simulink model "e11_pmsm_nonlin_fwc"  (R2024b)
settings: Solver=ode23tb  StartTime=0.0  StopTime=2  MaxStep=0.0001  RelTol=1e-3  EnableMultiTasking=on
InitFcn:
  | d = fileparts(mfilename('fullpath')); while ~exist(fullfile(d, 'models', 'matlab', 'mcb_e11_nonlin_setup.m'), 'file') up = fileparts(d); if strcmp(up, d), break; end, d = up; end, run(fullfile(d, 'models', 'matlab', 'mcb_e11_nonlin_setup.m'));
model workspace (MAT data in the model file):
  encoderResolution = 2000
  hallOffset = '0.5'
  indexOffset = 850
  polePairs = '4'
undefined symbols (not defined in the file): PI_params, pmsm, PU_System, PWM_frequency, Ts, Ts_motor, Ts_speed
libraries: nesl_utility x11, mcbcontrolslib x9, fl_lib x8, ee_lib x7, slpidlib x3, mcbpmsmnonlinearlib x3, mcbpositiondecoderlib x2, nesl_utility_internal x2, simulink x1, eeGeneralControl x1, mcbutilslib x1
(part 1 of 2)
settings Model: Creator=The MathWorks, Inc.  LastModifiedBy=xlin
settings SolverCC: AlgebraicLoopSolver=TrustRegion  MaxZcPerStep=1
settings DataIOCC: LimitDataPoints=on  SaveFormat=Array  SaveOutput=off  SaveTime=off  ReturnWorkspaceOutputs=off
settings OptimizationCC: DefaultParameterBehavior=Inlined  DefaultUnderspecifiedDataType=single  OptimizeBlockIOStorage=off  ReuseModelBlockBuffer=off  EnhancedBackFolding=on  ExpressionDepthLimit=2147483647  ZeroExternalMemoryAtStartup=off  InitFltsAndDblsToZero=on  NoFixptDivByZeroProtection=on  EfficientFloat2IntCast=on  EfficientMapNaN2IntZero=off  LifeSpan=Inf  MaxStackSize=64  DifferentSizesBufferReuse=on  EfficientTunableParamExpr=on
settings DebuggingCC: ReadBeforeWriteMsg=DisableAll  WriteAfterWriteMsg=DisableAll  WriteAfterReadMsg=DisableAll  CheckSSInitialOutputMsg=off  SignalResolutionControl=TryResolveAllWithWarning  SolverPrmCheckMsg=warning  InheritedTsInSrcMsg=none  MultiTaskDSMMsg=none  MultiTaskCondExecSysMsg=none  TasksWithSamePriorityMsg=none  SigSpecEnsureSampleTimeMsg=none  IntegerOverflowMsg=none  ParameterPrecisionLossMsg=none  FcnCallInpInsideContextMsg=warning  UnconnectedInputMsg=warning  UnconnectedOutputMsg=warning  UnconnectedLineMsg=warning  AllowSymbolicDim=off  StateNameClashWarn=warning  SFUnexpectedBacktrackingDiag=warning  SFNoUnconditionalDefaultTransitionDiag=warning  SFExecutionAtInitializationDiag=none  IntegerSaturationMsg=none  ArithmeticOperatorsInVariantConditions=warning
settings HardwareCC: TargetBitPerChar=16  TargetBitPerInt=16  TargetBitPerPointer=16  TargetLargestAtomicInteger=Integer  TargetIntDivRoundTo=Zero  TargetEndianess=LittleEndian  TargetWordSize=16  TargetHWDeviceType=TI C2000
settings ModelReferenceCC: EnableRefExpFcnMdlSchedulingChecks=on  ModelReferenceNumInstancesAllowed=Single  PropagateSignalLabelsOutOfModel=off
settings SFSimCC: SimUseLocalCustomCode=off  MATLABDynamicMemAlloc=off  CustomCodeUndefinedFunction=UseInterfaceOnly
settings RTWCC: Description=Embedded Coder  SystemTargetFile=ert.tlc  TemplateMakefile=ert_default_tmf  GenerateReport=on  RTWUseLocalCustomCode=off  CustomHeaderCode="#include \"F2837xD_Ipc_drivers.h\""  Toolchain=Texas Instruments Code Composer Studio (C2000)  LaunchReport=on  GPUComputeCapability=3.5  DLArmComputeVersion=19.05
settings CodeAppCC: ForceParamTrailComments=on  IgnoreCustomStorageClasses=off  OperatorAnnotations=on  SimulinkDataObjDesc=on  SFDataObjDesc=on  InsertBlockDesc=on  InternalIdentifier=Classic
settings ERTTargetCC: ExtModeStaticAlloc=on  ExtModeStaticAllocSize=10000  ERTCustomFileTemplate=example_file_process.tlc  SuppressUnreachableDefaultCases=off  DynamicArrayContainerType=coder::array
settings ConfigComp: CovMetricSettings=dw  CovSaveCumulativeToWorkspaceVar=on  CovSaveSingleToWorkspaceVar=on  CovExternalEMLEnable=off  CovSFcnEnable=off

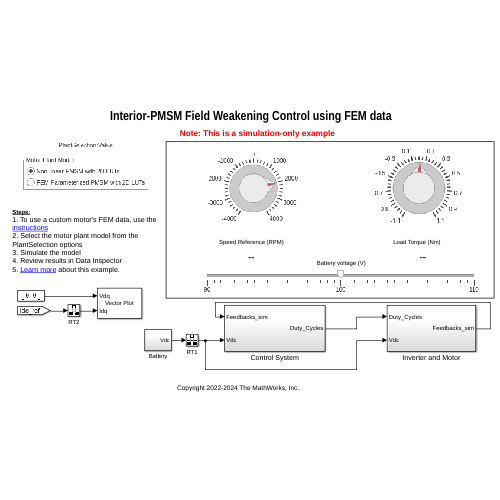
[thumbnail: Simulink's stored preview of the top-level diagram]
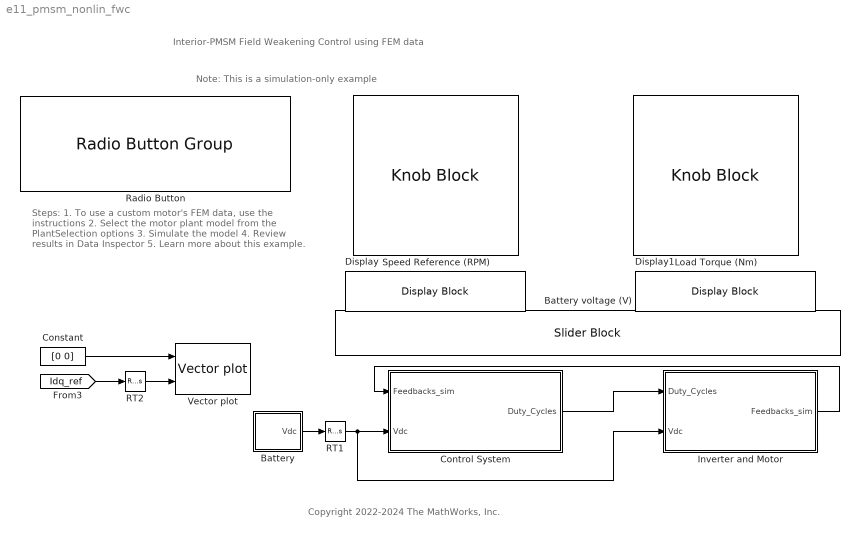
== system e11_pmsm_nonlin_fwc ==
  note: Steps:
      | 1. To use a custom motor's FEM data, use the instructions
      | 2. Select the motor plant model from the PlantSelection options
      | 3. Simulate the model
      | 4. Review results in Data Inspector
      | 5. Learn more about this example.
  note: Copyright 2022-2024 The MathWorks, Inc.
  note: Note: This is a simulation-only example
  note: Interior-PMSM Field Weakening Control using FEM data
  Battery : Subsystem
  Battery voltage (V) : SliderBlock  LabelPosition=Hide  ScaleMin=90  ScaleMax=110  TickInterval=10
  Constant : Constant  Value=[0 0]
  Control System : Subsystem
  Display : DisplayBlock  LabelPosition=Hide  Format=Integer  Transparency=1
  Display1 : DisplayBlock  LabelPosition=Hide  Transparency=1
  Inverter and Motor : Subsystem
  Load Torque (Nm) : KnobBlock  LabelPosition=Hide  ScaleMin=-1.1  ScaleMax=1.1
  RT1 : RateTransition  Deterministic=off  OutPortSampleTime=Ts
  RT2 : RateTransition  Deterministic=off  OutPortSampleTime=0.01
  Radio Button : RadioButtonGroup  SelectedLabel=Non-linear PMSM with 2D LUTs  ButtonGroupName=Motor Plant Model
      settings: Values={{'Non-linear PMSM with 2D LUTs', 'FEM Parameterized PMSM with 2D LUTs'}, [0 1]}
  Speed Reference (RPM) : KnobBlock  LabelPosition=Hide  ScaleMin=-4000  ScaleMax=4000
  Vector plot : mcbutilslib/Vector plot  InputSignals=Vdq Idq  ReferenceFrame=Rotating Reference Frame  axisAlign=D-axis  thetaUnits=Radians  angleUnits=Radians  OpenFigAtSimStart=off  debugEnable=0
      settings: LibrarySourceBlock=mcblib/Signal Management/Vector plot
  wires:
  Control System/1(Duty_Cycles) -> Inverter and Motor/1(Duty_Cycles)
  Constant/1 -> Vector plot/1
  [Idq_ref] -> RT2/1
  RT2/1 -> Vector plot/2
  Inverter and Motor/1(Feedbacks_sim) -> Control System/1(Feedbacks_sim)
  RT1/1 -> Inverter and Motor/2(Vdc), Control System/2(Vdc)
  Battery/1(Vdc) -> RT1/1

== system e11_pmsm_nonlin_fwc/Battery ==
  Battery Voltage : Constant  Value=100
  Vdc : Outport
  wires:
  Battery Voltage/1 -> Vdc/1

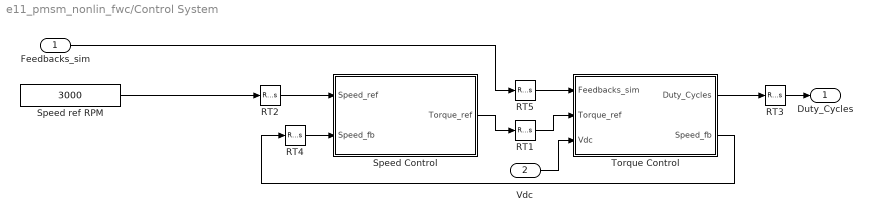
== system e11_pmsm_nonlin_fwc/Control System ==
  Feedbacks_sim : Inport
  Vdc : Inport  Port=2
  RT1 : RateTransition  Deterministic=off  OutPortSampleTime=Ts
  RT2 : RateTransition  Deterministic=off  OutPortSampleTime=Ts_speed
  RT3 : RateTransition  Deterministic=off
  RT4 : RateTransition  Deterministic=off  OutPortSampleTime=Ts_speed
  RT5 : RateTransition  Deterministic=off  OutPortSampleTime=Ts
  Speed Control : Subsystem  TreatAsAtomicUnit=on  SystemSampleTime=Ts_speed
      settings: RTWSystemCode=Nonreusable function
  Speed ref RPM : Constant  Value=3000  OutDataTypeStr=Inherit: Inherit via back propagation  SampleTime=-1
  Torque Control : Subsystem
      settings: RTWSystemCode=Nonreusable function
  Duty_Cycles : Outport
  wires:
  Feedbacks_sim/1 -> RT5/1
  Torque Control/2(Speed_fb) -> RT4/1
  RT1/1 -> Torque Control/2(Torque_ref)
  Speed Control/1(Torque_ref) -> RT1/1
  RT5/1 -> Torque Control/1(Feedbacks_sim)
  RT4/1 -> Speed Control/2(Speed_fb)
  Torque Control/1(Duty_Cycles) -> RT3/1
  RT2/1 -> Speed Control/1(Speed_ref)
  RT3/1 -> Duty_Cycles/1
  Vdc/1 -> Torque Control/3(Vdc)
  Speed ref RPM/1 -> RT2/1

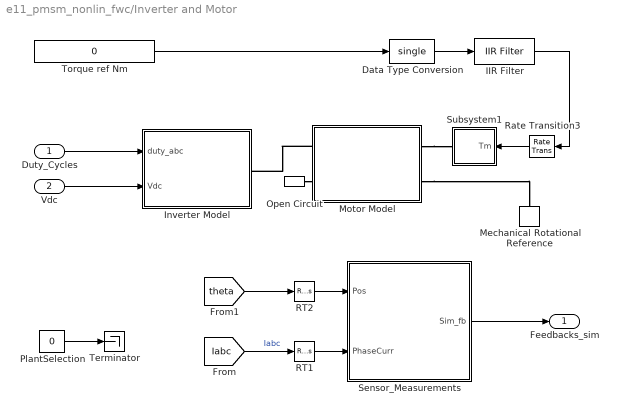
== system e11_pmsm_nonlin_fwc/Inverter and Motor ==
  Duty_Cycles : Inport
  Vdc : Inport  Port=2
  Data Type Conversion : DataTypeConversion  OutDataTypeStr=single  SaturateOnIntegerOverflow=off  RndMeth=Floor
  IIR Filter : mcbcontrolslib/IIR Filter  VariantControl=Low Pass Filter  VariantSelect=Low-pass  FilterConstantInputType=Specify via dialog  Filter_constant=0.01  advancedSettings=off  Ts=50e-6  cutOff_freq=32.1525
  Inverter Model : Subsystem
  Mechanical Rotational Reference : fl_lib/Mechanical/Rotational Elements/Mechanical Rotational Reference
  Motor Model : Subsystem  Variant=on
  Open Circuit : fl_lib/Electrical/Electrical Elements/Open Circuit  v_specify=off  v_priority=None  v=0 V  v_nominal_specify=off  v_nominal_value=1  v_nominal_unit=V
  PlantSelection : Constant  Value=0
  RT1 : RateTransition  Deterministic=off  OutPortSampleTime=Ts_simulink
  RT2 : RateTransition  Deterministic=off  OutPortSampleTime=Ts_simulink
  Rate Transition3 : RateTransition  Deterministic=off  OutPortSampleTime=Ts_motor
  Sensor_Measurements : Subsystem
  Subsystem1 : Subsystem
  Terminator : Terminator
  Torque ref Nm : Constant  Value=0  OutDataTypeStr=dataType  SampleTime=-1
  Feedbacks_sim : Outport  VectorParamsAs1DForOutWhenUnconnected=off
  wires:
  Sensor_Measurements/1(Sim_fb) -> Feedbacks_sim/1
  Torque ref Nm/1 -> Data Type Conversion/1
  Data Type Conversion/1 -> IIR Filter/1
  IIR Filter/1 -> Rate Transition3/1
  RT2/1 -> Sensor_Measurements/1(Pos)
  Rate Transition3/1 -> Subsystem1/1(Tm)
  [theta] -> RT2/1
  RT1/1 -> Sensor_Measurements/2(PhaseCurr)
  [Iabc] -> RT1/1  "Iabc"
  Duty_Cycles/1 -> Inverter Model/1(duty_abc)
  PlantSelection/1 -> Terminator/1
  Vdc/1 -> Inverter Model/2(Vdc)
  connections:
  Open Circuit/LConn1 -- Motor Model/LConn2
  Motor Model/RConn2 -- Mechanical Rotational Reference/LConn1
  Motor Model/RConn1 -- Subsystem1/RConn1
  Motor Model/LConn1 -- Inverter Model/RConn1

== system e11_pmsm_nonlin_fwc/Control System/Speed Control ==
  Speed_ref : Inport
  Speed_fb : Inport  Port=2
  PI_Controller_Speed : Subsystem
  rpm2pu : Subsystem
  Torque_ref : Outport  VectorParamsAs1DForOutWhenUnconnected=off
  wires:
  Speed_ref/1 -> rpm2pu/1(In1)  "speed_ref_rpm"
  Speed_fb/1 -> PI_Controller_Speed/2(Speed_fb)  "speed_fb"
  PI_Controller_Speed/1(T_ref) -> Torque_ref/1
  rpm2pu/1(Speed_ref) -> PI_Controller_Speed/1(Speed_ref)  "speed_ref"

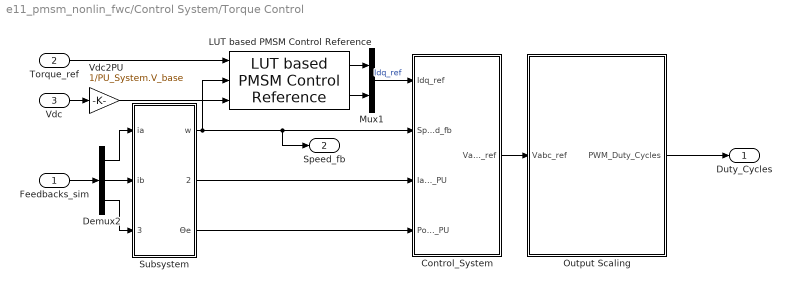
== system e11_pmsm_nonlin_fwc/Control System/Torque Control ==
  Feedbacks_sim : Inport
  Torque_ref : Inport  Port=2
  Vdc : Inport  Port=3
  Control_System : Subsystem
  Demux2 : Demux  Outputs=3
  LUT based PMSM Control Reference : mcbpmsmnonlinearlib/LUT based PMSM Control Reference  motorType=Interior PMSM  FWCMethod=CVCP  polePairs=pmsm.p  Rs=pmsm.Rs  nonLinearityChoice=Non-linear model with id and iq LUTs  Ld=pmsm.Ld  Lq=pmsm.Lq  FluxPM=pmsm.FluxPM  Vdc_input_select=Input port - use 2D LUT (scaled-w based)  vdc=inverter.V_dc  vdcVec=[18 30]  idVec=PMSMLUT.idVec  iqVec=PMSMLUT.iqVec  LdTable=PMSMLUT.LdTable  LqTable=PMSMLUT.LqTable  FluxPMTable=PMSMLUT.FluxPMTable  FluxDTable=[-1.6,-1.6,-1.6,-1.6,-1.6;2.4,2.4,2.4,2.4,2.4;6.4,6.4,6.4,6.4,6.4;10.4,10.4,10.4,10.4,10.4]*1e-3  FluxQTable=[-8,-4,0,4,8;-8,-4,0,4,8;-8,-4,0,4,8;-8,-4,0,4,8]*1e-3  useMeasTorqTable=off  MeasuredTorqTable=[-3.4560,-1.7280,0, 1.7280, 3.4560;-2.4960,-1.2480,0, 1.2480, 2.4960;-1.5360,-0.7680,0, 0.7680, 1.5360;-0.5760,-0.2880,0, 0.2880, 0.5760]  useTorquePct=off  CustomGrid=off  trefVec=PMSMLUT.trefVec  trefPctVec=[0 50 100]  Tenvelope=[0.3 0.3 0.15 0.05]  wrpmVec=PMSMLUT.wrpmVec  idTable=PMSMLUT.idTable  iqTable=PMSMLUT.iqTable  idTable3d=cat(3,[0,0,0,-7.1;-0.4579,-0.4579,-0.4579,-7.1;-1.4457,-1.4457,-1.4457,-7.1],[0,0,0,0;-0.4579,-0.4579,-0.4579,-1.2581;-1.4457,-1.4457,-1.4457,-4.5085])  iqTable3d=cat(3,[0,0,0,0;3.8539,3.8539,3.8539,0;6.9513,6.9513,6.9513,0],[0,0,0,0;3.8539,3.8539,3.8539,3.7611;6.9513,6.9513,6.9513,5.4848])  ilimit=maxMotorCurrent  Bv=pmsm.B  Units=Per-Unit (PU)  V_base=PU_System.V_base  I_base=PU_System.I_base  N_base=pmsm.N_base  T_base=0.74112  scaledTables=on  saveLUTs=off  useDefaultPlotOptions=on  RPM2plot=3000  Torque2plot=0.1  driveChar2plot=off  enableiMax2plot=off  imax2plot=10
      settings: LibrarySourceBlock=mcblib/Controls/Control Reference/LUT based PMSM Control Reference
  Mux1 : Mux  Inputs=2
  Output Scaling : Subsystem
  Subsystem : Subsystem
  Vdc2PU : Gain  Gain=1/PU_System.V_base  RndMeth=Simplest  OutDataTypeStr=Inherit: Same as input
  Duty_Cycles : Outport  InitialOutput=0  VectorParamsAs1DForOutWhenUnconnected=off
  Speed_fb : Outport  Port=2  InitialOutput=0  VectorParamsAs1DForOutWhenUnconnected=off
  wires:
  Control_System/1(Vabc_ref) -> Output Scaling/1(Vabc_ref)
  Output Scaling/1(PWM_Duty_Cycles) -> Duty_Cycles/1
  Feedbacks_sim/1 -> Demux2/1
  Subsystem/1(w) -> Speed_fb/1, Control_System/2(Speed_fb), LUT based PMSM Control Reference/2
  Demux2/1 -> Subsystem/1(ia)
  Demux2/2 -> Subsystem/2(ib)
  Demux2/3 -> Subsystem/3(pos_rad)
  Subsystem/2(iab_pu) -> Control_System/3(Iab_meas_PU)
  Subsystem/3(ϴe) -> Control_System/4(Pos_meas_PU)
  LUT based PMSM Control Reference/1 -> Mux1/1
  LUT based PMSM Control Reference/2 -> Mux1/2
  Mux1/1 -> Control_System/1(Idq_ref)  "Idq_ref"
  Torque_ref/1 -> LUT based PMSM Control Reference/1
  Vdc/1 -> Vdc2PU/1
  Vdc2PU/1 -> LUT based PMSM Control Reference/3

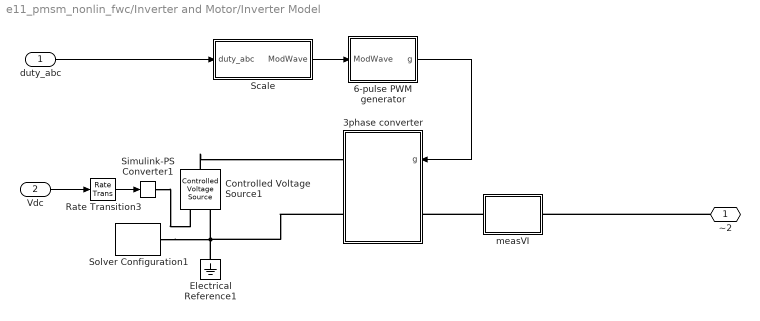
== system e11_pmsm_nonlin_fwc/Inverter and Motor/Inverter Model ==
  duty_abc : Inport
  Vdc : Inport  Port=2
  3phase converter : Subsystem
  6-pulse PWM generator : Subsystem  mask{fs=PWM_frequency}
      mask prompts: fs "Carrier Frequency (Hz)"
  Controlled Voltage Source1 : fl_lib/Electrical/Electrical Sources/Controlled Voltage Source
  Electrical Reference1 : fl_lib/Electrical/Electrical Elements/Electrical Reference
  Rate Transition3 : RateTransition  Deterministic=off  OutPortSampleTime=Ts_motor
  Scale : Subsystem
  Simulink-PS Converter1 : nesl_utility/Simulink-PS Converter  PhysicalDomain=network_engine_domain  SubClassName=ps_input  LeftPortType=input  RightPortType=output  PseudoPeriodic=off  Frequencies=[]  NoiseDistribution=none  NoiseParameters=[]  Unit=1  AffineConversion=off  FilteringAndDerivatives=provide  SimscapeFilterOrder=1  InputFilterTimeConstant=0.001  UdotUserProvided=0
  Solver Configuration1 : nesl_utility/Solver Configuration  PhysicalDomain=network_engine_domain  SubClassName=solver  LeftPortType=input  RightPortType=generic  Tones=[]  Harmonics=[]  SimulateNoise=off  Profile=off  UseLocalSampling=off  EnableSwitchedLinearOptims=on  FrequencyDomain=off  UseCCode=off  RelTol=0.001  AbsTol=0.001  MinStep=1e-09  ToWorkspace=off  RevertToSquareIcSolve=off  NumHomotopyIterations=100  PhasorMode=off  PhasorModeNumHarmonics=1  ConsistencySolver=NEWTON_XTOL_AFTER_FTOL  IndexReductionMethod=DerivativeReplacement  DoDC=off  ResidualTolerance=1e-09  ConsistencyTolSource=GLOBAL  ConsistencyAbsTol=0.001  ConsistencyRelTol=0.001  ConsistencyTolFactor=1e-09  UseLocalSolver=on  LocalSolverChoice=NE_BACKWARD_EULER_ADVANCER  ResolveIndetEquations=on  FunctionEvalNumThread=1  LocalSolverSampleTime=Ts_motor  DoFixedCost=on  MaxNonlinIter=1  MaxModeIter=2  ComputeImpulses=off  ImpulseIterations=2  LinearAlgebra=Sparse  LinearAlgebraNumThread=0  EquationFormulation=NE_TIME_EF  DelaysMemoryBudget=1024  AutomaticFiltering=off  FilteringTimeConstant=0.001  PartitionStorageMethod=AS_NEEDED  PartitionMemoryBudget=1024  PartitionMethod=ROBUST  MultibodyUseLocalSolver=off  MultibodyLocalSolverChoice=ODE1  MultibodyLocalSolverSampleTime=0.001
  measVI : Subsystem
  ~2 : PMIOPort  Side=Right
  wires:
  6-pulse PWM generator/1(g) -> 3phase converter/1(g)
  duty_abc/1 -> Scale/1(duty_abc)
  Scale/1(ModWave) -> 6-pulse PWM generator/1(ModWave)
  Rate Transition3/1 -> Simulink-PS Converter1/1
  Vdc/1 -> Rate Transition3/1
  connections:
  measVI/LConn1 -- 3phase converter/LConn1
  Electrical Reference1/LConn1 -- Solver Configuration1/RConn1 -- 3phase converter/RConn2 -- Controlled Voltage Source1/RConn2
  Controlled Voltage Source1/LConn1 -- 3phase converter/RConn1
  ~2/RConn1 -- measVI/RConn1
  Simulink-PS Converter1/RConn1 -- Controlled Voltage Source1/RConn1

== system e11_pmsm_nonlin_fwc/Inverter and Motor/Motor Model ==
  FEM Parameterized PMSM 2D LUTs : Subsystem  VariantControl=(get_param([bdroot '/Inverter and Motor/PlantSelection'], 'Value') == '1')
  Non-linear PMSM with 2D LUTs : Subsystem  VariantControl=(get_param([bdroot '/Inverter and Motor/PlantSelection'], 'Value') == '0')
  ~ : PMIOPort  Side=Left
  neutral : PMIOPort  Port=2  Side=Left
  R : PMIOPort  Port=3  Side=Right
  C : PMIOPort  Port=4  Side=Right

== system e11_pmsm_nonlin_fwc/Inverter and Motor/Sensor_Measurements ==
  Pos : Inport
  PhaseCurr : Inport  Port=2
  Data Type Conversion2 : DataTypeConversion  OutDataTypeStr=single  RndMeth=Simplest  SaturateOnIntegerOverflow=off
  Data Type Conversion4 : DataTypeConversion  OutDataTypeStr=single  RndMeth=Simplest  SaturateOnIntegerOverflow=off
  Delay1 : Delay  DelayLength=PI_params.delay_Currents
  Delay2 : Delay  DelayLength=PI_params.delay_Position
  Mux2 : Mux  Inputs=2
  Selector : Selector  InputPortWidth=3  IndexOptions=Index vector (dialog)  Indices=[1 2]  OutputSizes=1
  Sim_fb : Outport  VectorParamsAs1DForOutWhenUnconnected=off
  wires:
  Delay1/1 -> Selector/1  "Iab_fb"
  Data Type Conversion4/1 -> Delay1/1
  PhaseCurr/1 -> Data Type Conversion4/1
  Pos/1 -> Data Type Conversion2/1
  Data Type Conversion2/1 -> Delay2/1  "Theta_m"
  Selector/1 -> Mux2/1
  Delay2/1 -> Mux2/2  "Theta_m"
  Mux2/1 -> Sim_fb/1

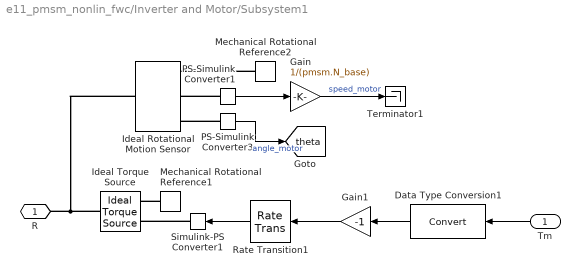
== system e11_pmsm_nonlin_fwc/Inverter and Motor/Subsystem1 ==
  Tm : Inport
  Data Type Conversion1 : DataTypeConversion  SaturateOnIntegerOverflow=off  RndMeth=Floor
  Gain : Gain  Gain=1/(pmsm.N_base)
  Gain1 : Gain  Gain=-1
  Ideal Rotational Motion Sensor : fl_lib/Mechanical/Mechanical Sensors/Ideal Rotational Motion Sensor  reference=foundation.enum.MeasurementReference.difference  acceleration_port=false  velocity_port=true  position_port=true  wrap_angle=simscape.enum.onoff.off  offset=0 rad
  Ideal Torque Source : fl_lib/Mechanical/Mechanical Sources/Ideal Torque Source
  Mechanical Rotational Reference1 : fl_lib/Mechanical/Rotational Elements/Mechanical Rotational Reference
  Mechanical Rotational Reference2 : fl_lib/Mechanical/Rotational Elements/Mechanical Rotational Reference
  PS-Simulink Converter1 : nesl_utility/PS-Simulink Converter  PhysicalDomain=network_engine_domain  SubClassName=ps_output  LeftPortType=input  RightPortType=output  PseudoPeriodic=off  Frequencies=[]  VectorFormat=inherit  Unit=inherit  AffineConversion=off
  PS-Simulink Converter3 : nesl_utility/PS-Simulink Converter  PhysicalDomain=network_engine_domain  SubClassName=ps_output  LeftPortType=input  RightPortType=output  PseudoPeriodic=off  Frequencies=[]  VectorFormat=inherit  Unit=inherit  AffineConversion=off
  Rate Transition1 : RateTransition
  Simulink-PS Converter1 : nesl_utility/Simulink-PS Converter  PhysicalDomain=network_engine_domain  SubClassName=ps_input  LeftPortType=input  RightPortType=output  PseudoPeriodic=off  Frequencies=[]  NoiseDistribution=none  NoiseParameters=[]  Unit=1  AffineConversion=off  FilteringAndDerivatives=provide  SimscapeFilterOrder=1  InputFilterTimeConstant=0.001  UdotUserProvided=0
  Terminator1 : Terminator
  "R " : PMIOPort  Side=Right
  tag scope: theta=global
  wires:
  Gain1/1 -> Rate Transition1/1
  Rate Transition1/1 -> Simulink-PS Converter1/1
  Data Type Conversion1/1 -> Gain1/1
  Tm/1 -> Data Type Conversion1/1
  PS-Simulink Converter1/1 -> Gain/1
  Gain/1 -> Terminator1/1  "speed_motor"
  PS-Simulink Converter3/1 -> [theta]  "angle_motor"
  connections:
  Mechanical Rotational Reference1/LConn1 -- Ideal Torque Source/RConn2
  Simulink-PS Converter1/RConn1 -- Ideal Torque Source/RConn1
  Ideal Torque Source/LConn1 -- Ideal Rotational Motion Sensor/LConn1 -- "R "/RConn1
  PS-Simulink Converter1/LConn1 -- Ideal Rotational Motion Sensor/RConn2
  PS-Simulink Converter3/LConn1 -- Ideal Rotational Motion Sensor/RConn3
  Mechanical Rotational Reference2/LConn1 -- Ideal Rotational Motion Sensor/RConn1

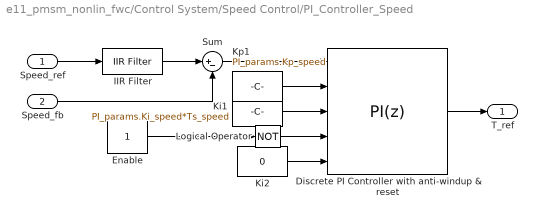
== system e11_pmsm_nonlin_fwc/Control System/Speed Control/PI_Controller_Speed ==
  Speed_ref : Inport
  Speed_fb : Inport  Port=2
  Discrete PI Controller with anti-windup & reset : slpidlib/PID Controller  Controller=PI  Form=Parallel  TimeDomain=Discrete-time  UseExternalTs=off  SampleTime=-1  IntegratorMethod=Forward Euler  FilterMethod=Forward Euler  ControllerParametersSource=external  P=1  I=1  UseKiTs=on  D=0  UseExternalDerivativeSource=off  N=100  UseFilter=on  TunerSelectOption=Transfer Function Based (PID Tuner App)  InitialConditionSource=external  InitialConditionForIntegrator=0  InitialConditionForFilter=0  DifferentiatorICPrevScaledInput=0  ExternalReset=level  TrackingMode=off  Kt=1  LimitOutput=on  SatLimitsSource=internal  UpperSaturationLimit=1  LowerSaturationLimit=-1  LinearizeAsGain=on  AntiWindupMode=clamping  Kb=1  LimitIntegrator=off  UpperIntegratorSaturationLimit=inf  LowerIntegratorSaturationLimit=-inf  RndMeth=Simplest  POutMin=[]  POutMax=[]  IOutMin=[]  IOutMax=[]  DOutMin=[]  DOutMax=[]  NOutMin=[]  NOutMax=[]  SumOutMin=[]  SumOutMax=[]  SaturationOutDataTypeStr=Inherit: Inherit via back propagation  SaturationOutMin=[]  SaturationOutMax=[]  PParamMin=[]  PParamMax=[]  IParamMin=[]  IParamMax=[]  DParamMin=[]  DParamMax=[]  NParamMin=[]  NParamMax=[]  KbParamMin=[]  KbParamMax=[]  KtParamMin=[]  KtParamMax=[]  KbOutMin=[]  KbOutMax=[]  KtOutMin=[]  KtOutMax=[]  IntegratorOutMin=[]  IntegratorOutMax=[]  FilterOutMin=[]  FilterOutMax=[]  SumI1OutMin=[]  SumI1OutMax=[]  SumI2OutMin=[]  SumI2OutMax=[]  SumI3OutMin=[]  SumI3OutMax=[]  SumI4OutMin=[]  SumI4OutMax=[]  SumDOutMin=[]  SumDOutMax=[]  DifferentiatorOutMin=[]  DifferentiatorOutMax=[]  FilterDiffOutCoefMin=[]  FilterDiffOutCoefMax=[]  ReciprocalOutMin=[]  ReciprocalOutMax=[]  SumDenOutMin=[]  SumDenOutMax=[]  SumNumOutMin=[]  SumNumOutMax=[]  DivideOutMin=[]  DivideOutMax=[]  UdiffTsProdOutMin=[]  UdiffTsProdOutMax=[]  NTsProdOutMin=[]  NTsProdOutMax=[]  UintegralTsProdOutMin=[]  UintegralTsProdOutMax=[]  UngainTsProdOutMin=[]  UngainTsProdOutMax=[]  ClampingZeroOutDataTypeStr=Inherit: Inherit via back propagation  ClampingZeroOutMin=[]  ClampingZeroOutMax=[]  FilterDenConstantOutDataTypeStr=Inherit: Inherit via back propagation  FilterDenConstantOutMin=[]  FilterDenConstantOutMax=[]  PCopyOutDataTypeStr=Inherit: Inherit via back propagation  PCopyOutMin=[]  PCopyOutMax=[]  NCopyOutDataTypeStr=Inherit: Inherit via back propagation  NCopyOutMin=[]  NCopyOutMax=[]  IntegratorContinuousStateAttributes=''  IntegratorStateMustResolveToSignalObject=off  IntegratorRTWStateStorageClass=Auto  FilterContinuousStateAttributes=''  FilterStateMustResolveToSignalObject=off  FilterRTWStateStorageClass=Auto  ParallelPVariant=ExternalParameters  IdealPVariant=Disabled  IVariant=ExternalParameters  DVariant=Disabled  IntegratorVariant=Discrete  SatVariant=Enabled  AWVariant=DiscClampingParallel  PCopyVariant=Disabled  TRVariant=Disabled  FdbkBlocksVariant=Forward  IdealPFdbkVariant=Disabled  SatFdbkVariant=Disabled  DerivativeFilterVariant=Disabled  NVariant=Disabled  NCopyVariant=Disabled_SignalSpec  FilterICVariant=Disabled  IntegratorICVariant=ExternalICs  ExternalResetVariant=ExternalReset  TRSumVariant=Passthrough  SumFdbkVariant=Disabled  SumVariant=Sum_PI  TsampFilterVariant=InternalTs  TsampNgainVariant=Passthrough  TsampIntegralVariant=Disabled_SignalSpec  ExternalSaturationOutDataTypeStr=Inherit: Same as second input  DerivativeSourceVariant=Disabled  PreIntVariant=InternalPreInt
  Enable : Constant  OutDataTypeStr=boolean  SampleTime=-1
  IIR Filter : mcbcontrolslib/IIR Filter  VariantControl=Low Pass Filter  VariantSelect=Low-pass  FilterConstantInputType=Specify via dialog  Filter_constant=0.1  advancedSettings=off  Ts=50e-6  cutOff_freq=353.6777
  Ki1 : Constant  Value=PI_params.Ki_speed*Ts_speed  OutDataTypeStr=dataType  SampleTime=-1
  Ki2 : Constant  Value=0  OutDataTypeStr=dataType  SampleTime=-1
  Kp1 : Constant  Value=PI_params.Kp_speed  OutDataTypeStr=dataType  SampleTime=-1
  Logical Operator : Logic  Operator=NOT  IconShape=distinctive  AllPortsSameDT=off  OutDataTypeStr=boolean
  Sum : Sum  Inputs=|+-
  T_ref : Outport  VectorParamsAs1DForOutWhenUnconnected=off
  wires:
  Discrete PI Controller with anti-windup & reset/1 -> T_ref/1
  Ki1/1 -> Discrete PI Controller with anti-windup & reset/3
  Kp1/1 -> Discrete PI Controller with anti-windup & reset/2
  Speed_fb/1 -> Sum/2
  Sum/1 -> Discrete PI Controller with anti-windup & reset/1
  Logical Operator/1 -> Discrete PI Controller with anti-windup & reset/4
  Enable/1 -> Logical Operator/1
  Ki2/1 -> Discrete PI Controller with anti-windup & reset/5
  Speed_ref/1 -> IIR Filter/1
  IIR Filter/1 -> Sum/1

== system e11_pmsm_nonlin_fwc/Control System/Speed Control/rpm2pu ==
  In1 : Inport
  Data Type Conversion2 : DataTypeConversion  OutDataTypeStr=dataType  RndMeth=Simplest  SaturateOnIntegerOverflow=off
  rpm2PU : Gain  Gain=1/pmsm.N_base  RndMeth=Simplest  OutDataTypeStr=Inherit: Same as input
  Speed_ref : Outport
  wires:
  Data Type Conversion2/1 -> Speed_ref/1
  rpm2PU/1 -> Data Type Conversion2/1
  In1/1 -> rpm2PU/1

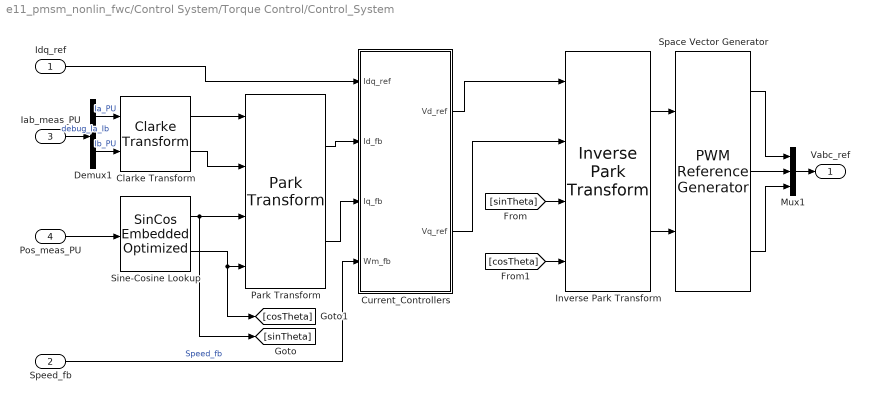
== system e11_pmsm_nonlin_fwc/Control System/Torque Control/Control_System ==
  Idq_ref : Inport
  Speed_fb : Inport  Port=2
  Iab_meas_PU : Inport  Port=3
  Pos_meas_PU : Inport  Port=4
  Clarke Transform : mcbcontrolslib/Clarke Transform  VariantControl=Variant2  PhaseInput=Two inputs  EnPowerInv=off
  Current_Controllers : Subsystem
  Demux1 : Demux  Outputs=2
  Inverse Park Transform : mcbcontrolslib/Inverse Park Transform  PhaseInput=Two inputs  AxisAlignment=D-axis  ThetaInput=Sine and Cosine electrical position  AngleInput=Per-unit  N_points=1024
  Mux1 : Mux  Inputs=3
  Park Transform : mcbcontrolslib/Park Transform  PhaseInput=Two inputs  AxisAlignment=D-axis  ThetaInput=Sine and Cosine electrical position  AngleInput=Per-unit  N_points=1024
  Sine-Cosine Lookup : mcbcontrolslib/SinCos Embedded Optimized  LabelModeActiveChoice=MCB_Sin  OptforProc=off  ApproximationMethod=None  UserApproxMethod=Lookup  ApproxStatus=None  InterpMethod=Linear point-slope  NumberOfDataPoints=16  NumberOfIterations=11  RemoveProtectionAgainstOutOfRangeInput=off  TableDataTypeStr=Inherit: Inherit via input  AngleInput=Per-unit  ThetaDataType=single  N_points=1024  DatatypeInput=Inherit from input  Datatype=single
  Space Vector Generator : mcbcontrolslib/PWM Reference Generator  inSignal=Valphabeta  modType=SVM: space vector modulation
  Vabc_ref : Outport  VectorParamsAs1DForOutWhenUnconnected=off
  wires:
  Park Transform/1 -> Current_Controllers/2(Id_fb)
  Park Transform/2 -> Current_Controllers/3(Iq_fb)
  Inverse Park Transform/1 -> Space Vector Generator/1
  Inverse Park Transform/2 -> Space Vector Generator/2
  Sine-Cosine Lookup/1 -> [sinTheta], Park Transform/3
  Sine-Cosine Lookup/2 -> [cosTheta], Park Transform/4
  [cosTheta] -> Inverse Park Transform/4
  [sinTheta] -> Inverse Park Transform/3
  Clarke Transform/2 -> Park Transform/2
  Clarke Transform/1 -> Park Transform/1
  Idq_ref/1 -> Current_Controllers/1(Idq_ref)
  Space Vector Generator/1 -> Mux1/1
  Space Vector Generator/2 -> Mux1/2
  Current_Controllers/1(Vd_ref) -> Inverse Park Transform/1
  Current_Controllers/2(Vq_ref) -> Inverse Park Transform/2
  Space Vector Generator/3 -> Mux1/3
  Mux1/1 -> Vabc_ref/1
  Demux1/1 -> Clarke Transform/1  "Ia_PU"
  Demux1/2 -> Clarke Transform/2  "Ib_PU"
  Iab_meas_PU/1 -> Demux1/1  "debug_Ia_Ib"
  Speed_fb/1 -> Current_Controllers/4(Wm_fb)  "Speed_fb"
  Pos_meas_PU/1 -> Sine-Cosine Lookup/1

== system e11_pmsm_nonlin_fwc/Control System/Torque Control/Output Scaling ==
  Vabc_ref : Inport
  Constant : Constant  Value=0.5  OutDataTypeStr=dataType  SampleTime=-1
  One_by_Two : Gain  Gain=0.5  RndMeth=Simplest  OutDataTypeStr=Inherit: Same as input
  Sum : Sum  Inputs=|++
  PWM_Duty_Cycles : Outport
  wires:
  Constant/1 -> Sum/2
  Vabc_ref/1 -> One_by_Two/1
  Sum/1 -> PWM_Duty_Cycles/1
  One_by_Two/1 -> Sum/1

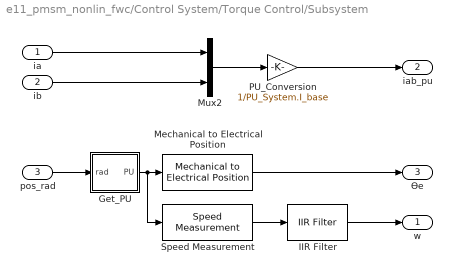
== system e11_pmsm_nonlin_fwc/Control System/Torque Control/Subsystem ==
  ia : Inport
  ib : Inport  Port=2
  pos_rad : Inport  Port=3
  "Get_PU " : Subsystem
  IIR Filter : mcbcontrolslib/IIR Filter  VariantControl=Low Pass Filter  VariantSelect=Low-pass  FilterConstantInputType=Specify via dialog  Filter_constant=IIR_filter_speed.coeff_Ts  advancedSettings=off  Ts=50e-6  cutOff_freq=1
  Mechanical to Electrical Position : mcbpositiondecoderlib/Mechanical to Electrical Position  PolePairsInputType=Specify via dialog  NrPP=pmsm.p  selectedRange=Per unit  MechOfstInputType=Specify via dialog  mechOffsetIn=0  maxAngleIn=1  InputDataType=dataType  VariantSelect=floating-point
  Mux2 : Mux  Inputs=2
  PU_Conversion : Gain  Gain=1/PU_System.I_base  RndMeth=Simplest  OutDataTypeStr=Inherit: Same as input
  Speed Measurement : mcbpositiondecoderlib/Speed Measurement  PositionUnit=Per unit  PositionScalingDatatype=uint32  SpeedCalculationMode=Time interval for speed calculation  SampleTimeAsync=Ts  MaximumApplicationSpeed=6000  SpeedResolution=5e-6  DelayLength=20  MaximumMeasurableSpeed=-0.98352  MeasurableSpeedResolution=7.6757e-12  SpeedUnit=Per unit based on dialog  PerUnitSpeed=PU_System.N_base  SpeedDataType=dataType
  w : Outport
  iab_pu : Outport  Port=2
  ϴe : Outport  Port=3
  wires:
  ib/1 -> Mux2/2
  "Get_PU "/1(PU) -> Speed Measurement/1, Mechanical to Electrical Position/1
  ia/1 -> Mux2/1
  PU_Conversion/1 -> iab_pu/1
  Speed Measurement/1 -> IIR Filter/1
  Mux2/1 -> PU_Conversion/1
  pos_rad/1 -> "Get_PU "/1(rad)
  IIR Filter/1 -> w/1
  Mechanical to Electrical Position/1 -> ϴe/1

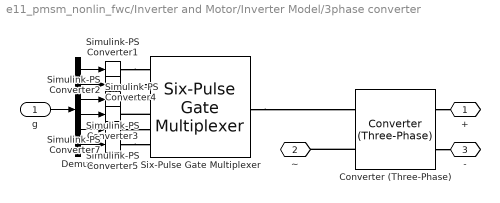
== system e11_pmsm_nonlin_fwc/Inverter and Motor/Inverter Model/3phase converter ==
  g : Inport
  Converter (Three-Phase) : ee_lib/Semiconductors & Converters/Converters/Converter (Three-Phase)  port_option=ee.enum.threePhasePort.composite  fidelity_option=ee.enum.converters.fidelity.detailed  device_type=ee.enum.converters.switchingdevice.ideal  showThermalPort=false  K=0  Vth=0.5 V  Vgt=1 V  Vgt_off=-1 V  Ih=1 A  Vf=0.8 V  Ron=0.001 Ohm  Rds=0.001 Ohm  Goff=1e-6 1/Ohm  Eon_scalar=22.86e-3 J  Eoff_scalar=17.14e-3 J  Eoff_natural_commutation=10e-3 J  Voff=300 V  Iout_scalar=600 A  onCurrentMeasDelay=0 s  useCurrentFromPreviousCycle=false  useVoltageFromPreviousCycle=false  diode_param=ee.enum.converters.protectiondiode.none  diode_Vf=0.8 V  diode_Ron=0.001 Ohm  diode_Goff=1e-5 1/Ohm  diode_C=50 nF  diode_iRM=-235 A  diode_iF=300 A  diode_idot=-50 A/us  diode_trr_param=ee.enum.converters.diodetrr.trr_factor  diode_trr_factor=3  diode_trr=15 us  diode_Qrr=1500 s*uA  diode_rec_loss_model=ee.enum.diode.reverseRecoveryModel.fixed  diode_ErecVal=0 J  diode_scaleWithIandV=false  diode_ErecMat=zeros(2, 3) J  diode_TjrecVec=[298.15, 398.15] K  diode_IfrecVec=[.1, 1, 10] A  diode_IrecVal=10 A  diode_VrecVal=10 V  diode_tFilter=1 / 1000 / 100 s  thermal_network_parameterization=ee.enum.thermalNetworkTopology.external  Rth=[.08, .5] K/W  Rth_Cauer=[.08, .1, .5] K/W  Rth_Foster=[.08, .14, .22, .16] K/W  thermal_mass_parameterization=ee.enum.thermalNetwork.timeconstant  thermal_mass=[.01, .5] J/K  thermal_mass_Cauer=[.01, .1, .5] J/K  thermal_mass_Foster=[.001, .005, .05, .5] J/K  thermal_time_constant=[.001, .2] s  thermal_time_constant_Cauer=[.001, .1, .2] s  thermal_time_constant_Foster=[7e-05, .0007, .01, .08] s  thermal_mass_initial_temperatures=[25, 25] degC  thermal_mass_initial_temperatures_Cauer=[25, 25, 25] degC  junction_thermal_mass=0.01 J/K  Tvec_initial_Foster=[25, 25, 25, 25] degC  snubber_type=ee.enum.converters.snubber.exclude  Cs=1e-7 F  Rs=0.1 Ohm  Vce_loss=[0, 150, 300] V
  Demux : Demux  Outputs=6
  Simulink-PS Converter{1..5,7} (6 alike) : nesl_utility/Simulink-PS Converter  PhysicalDomain=network_engine_domain  SubClassName=ps_input  LeftPortType=input  RightPortType=output  PseudoPeriodic=off  Frequencies=[]  NoiseDistribution=none  NoiseParameters=[]  Unit=1  AffineConversion=off  FilteringAndDerivatives=provide  SimscapeFilterOrder=1  InputFilterTimeConstant=0.001  UdotUserProvided=0
  Six-Pulse Gate Multiplexer : ee_lib/Semiconductors & Converters/Converters/Six-Pulse Gate Multiplexer  port_option=ee.enum.controlport.ps
  + : PMIOPort  Side=Right
  ~ : PMIOPort  Port=2  Side=Left
  - : PMIOPort  Port=3  Side=Right
  wires:
  g/1 -> Demux/1
  Demux/1 -> Simulink-PS Converter1/1
  Demux/2 -> Simulink-PS Converter2/1
  Demux/3 -> Simulink-PS Converter3/1
  Demux/4 -> Simulink-PS Converter4/1
  Demux/6 -> Simulink-PS Converter7/1
  Demux/5 -> Simulink-PS Converter5/1
  connections:
  Simulink-PS Converter1/RConn1 -- Six-Pulse Gate Multiplexer/LConn1
  Converter (Three-Phase)/RConn2 -- -/RConn1
  Converter (Three-Phase)/RConn1 -- +/RConn1
  Converter (Three-Phase)/LConn2 -- ~/RConn1
  Six-Pulse Gate Multiplexer/RConn1 -- Converter (Three-Phase)/LConn1
  Simulink-PS Converter2/RConn1 -- Six-Pulse Gate Multiplexer/LConn2
  Simulink-PS Converter3/RConn1 -- Six-Pulse Gate Multiplexer/LConn3
  Six-Pulse Gate Multiplexer/LConn4 -- Simulink-PS Converter4/RConn1
  Simulink-PS Converter5/RConn1 -- Six-Pulse Gate Multiplexer/LConn5
  Simulink-PS Converter7/RConn1 -- Six-Pulse Gate Multiplexer/LConn6

== system e11_pmsm_nonlin_fwc/Inverter and Motor/Inverter Model/6-pulse PWM generator ==
  ModWave : Inport
  Data Type Conversion : DataTypeConversion  SaturateOnIntegerOverflow=off  RndMeth=Floor
  Mux : Mux  Inputs=2
  NOT : Logic  Operator=NOT  IconShape=distinctive  AllPortsSameDT=off  OutDataTypeStr=boolean
  Relay : Relay
  Repeating Sequence Interpolated : simulink/Sources/Repeating Sequence Interpolated  OutValues=[0 1 0 -1 0].'  TimeValues=0.25/fs*[0 1 2 3 4].'  LookUpMeth=Interpolation-Use End Values  tsamp=Ts_motor  OutMin=[]  OutMax=[]  OutDataTypeStr=double  OutputDataTypeScalingMode=double  OutDataType=fixdt(0,8)  OutScaling=2^-10
  Selector : Selector  InputPortWidth=6  IndexOptions=Index vector (dialog)  Indices=[1 4 2 5 3 6]  OutputSizes=1
  Sum : Sum  Inputs=|+-
  g : Outport
  wires:
  Selector/1 -> g/1
  Mux/1 -> Selector/1
  Repeating Sequence Interpolated/1 -> Sum/2  "carrier"
  Sum/1 -> Relay/1
  Relay/1 -> Mux/1, NOT/1
  NOT/1 -> Data Type Conversion/1
  ModWave/1 -> Sum/1
  Data Type Conversion/1 -> Mux/2

== system e11_pmsm_nonlin_fwc/Inverter and Motor/Inverter Model/Scale ==
  duty_abc : Inport
  Constant : Constant  Value=-0.5  OutDataTypeStr=double  SampleTime=Ts_motor
  Data Type Conversion : DataTypeConversion  OutDataTypeStr=double  RndMeth=Simplest  SaturateOnIntegerOverflow=off
  Gain : Gain  Gain=2
  Sum : Sum  Inputs=|++
  ModWave : Outport
  wires:
  Sum/1 -> Gain/1
  Constant/1 -> Sum/2
  duty_abc/1 -> Data Type Conversion/1
  Gain/1 -> ModWave/1  "ModWave"
  Data Type Conversion/1 -> Sum/1

== system e11_pmsm_nonlin_fwc/Inverter and Motor/Inverter Model/measVI ==
  Current Sensor (Three-Phase) : ee_lib/Sensors & Transducers/Current Sensor (Three-Phase)
  Line Voltage Sensor (Three-Phase) : ee_lib/Sensors & Transducers/Line Voltage Sensor (Three-Phase)
  Low-Pass Filter (Discrete or Continuous) : eeGeneralControl/Low-Pass Filter (Discrete or Continuous)  K=1  T=5e-4  B=inf  A=-inf  init_option=Inherited from block input  x0=0  Ts=-1
  PS-Simulink Converter2 : nesl_utility_internal/PS-Simulink Converter  PhysicalDomain=network_engine_domain  SubClassName=ps_output  LeftPortType=input  RightPortType=output  PseudoPeriodic=off  Frequencies=[]  VectorFormat=1-D array  Unit=inherit  AffineConversion=off
  PS-Simulink Converter3 : nesl_utility_internal/PS-Simulink Converter  PhysicalDomain=network_engine_domain  SubClassName=ps_output  LeftPortType=input  RightPortType=output  PseudoPeriodic=off  Frequencies=[]  VectorFormat=1-D array  Unit=inherit  AffineConversion=off
  Terminator : Terminator
  ~1 : PMIOPort  Side=Left
  ~2 : PMIOPort  Port=2  Side=Right
  tag scope: Iabc=global
  wires:
  PS-Simulink Converter2/1 -> Low-Pass Filter (Discrete or Continuous)/1  "Vabc"
  PS-Simulink Converter3/1 -> [Iabc]  "Iabc"
  Low-Pass Filter (Discrete or Continuous)/1 -> Terminator/1
  connections:
  Current Sensor (Three-Phase)/RConn1 -- PS-Simulink Converter3/LConn1
  PS-Simulink Converter2/LConn1 -- Line Voltage Sensor (Three-Phase)/RConn1
  Current Sensor (Three-Phase)/RConn2 -- ~2/RConn1
  Line Voltage Sensor (Three-Phase)/LConn1 -- ~1/RConn1 -- Current Sensor (Three-Phase)/LConn1

== system e11_pmsm_nonlin_fwc/Inverter and Motor/Motor Model/FEM Parameterized PMSM 2D LUTs ==
  FEM-Parameterized PMSM : ee_lib/Electromechanical/Permanent Magnet/FEM-Parameterized PMSM  parameterization=2  winding_type=ee.enum.statorconnection.wye  iVec=[-2, 0, 2] A  xVec=[0, 20, 40, 60] deg  dfluxdiMatrix=0.0002 * ones(3, 4) Wb/A  dfluxdxMatrix=[0, -.16, .16, 0; 0, -.16, .16, 0; 0, -.16, .16, 0] Wb/rad  calculate_torque_matrix=1  TorqueMatrix=zeros(3, 3, 3, 4) N*m  idVec1=PMSMLUT.idVec A  iqVec1=PMSMLUT.iqVec A  LdMatrix=PMSMLUT.LdTable H  LqMatrix=PMSMLUT.LqTable H  PmMatrix=PMSMLUT.FluxPMTable Wb  interp_method=simscape.enum.interpolation.linear  N=pmsm.p  Rs=pmsm.Rs Ohm  Ms=0.00002 H  L0=0.00016 H  loss_param=ee.enum.fem_motor.ironLossesExtended.none  losses_oc=[0, 0, 0] W  losses_sc=[0, 0, 0] W  f_losses=10000 Hz  Isc_losses=10000 A  Inertia=pmsm.J kg*m^2  lam=pmsm.B N*m/(rad/s)  i_d_specify=off  i_d_priority=High  i_d=0 A  i_d_nominal_specify=off  i_d_nominal_value=1  i_d_nominal_unit=A  i_q_specify=off  i_q_priority=High  i_q=0 A  i_q_nominal_specify=off  i_q_nominal_value=1  i_q_nominal_unit=A  torque_specify=off  torque_priority=None  torque=0 N*m  torque_nominal_specify=off  torque_nominal_value=1  torque_nominal_unit=N*m  angular_velocity_specify=on  angular_velocity_priority=None  angular_velocity=100 rpm  angular_velocity_nominal_specify=off  angular_velocity_nominal_value=1  angular_velocity_nominal_unit=rpm  angular_position_specify=on  angular_position_priority=None  angular_position=0 deg  angular_position_nominal_specify=off  angular_position_nominal_value=1  angular_position_nominal_unit=deg  alpha=3.93e-3 1/K  alpha_flux=-0.001 1/K  Tmeas=298.15 K  stator_thermal_mass=100 J/K  stator_initial_temperatures=[298.15, 298.15, 298.15] K  rotor_thermal_mass=200 J/K  rotor_initial_temperature=298.15 K  Rm_percent_rotor=90  Rd_percent_rotor=30  idVec=[-200, 0, 200] A  iqVec=[-200, 0, 200] A  dfluxAdiaMatrix3D=zeros(3, 3, 4) Wb/A  dfluxAdibMatrix3D=zeros(3, 3, 4) Wb/A  dfluxAdicMatrix3D=zeros(3, 3, 4) Wb/A  dfluxAdxMatrix3D=zeros(3, 3, 4) Wb/rad  TorqueMatrix3D=zeros(3, 3, 4) N*m  iaVec=[-200, 0, 200] A  ibVec=[-200, 0, 200] A  icVec=[-200, 0, 200] A  dfluxAdiaMatrix=zeros(3, 3, 3, 4) Wb/A  dfluxAdibMatrix=zeros(3, 3, 3, 4) Wb/A  dfluxAdicMatrix=zeros(3, 3, 3, 4) Wb/A  dfluxAdxMatrix=zeros(3, 3, 3, 4) Wb/rad  param_dq0=ee.enum.fem_motor.fluxTabulationOption.DQcartesian  winding_type_dq0=ee.enum.statorconnection.wye  expose_neutral_port=ee.enum.fem_motor.exposeNeutralPort.no  nPolePairs=4  parks_type=ee.enum.fem_motor.parksType.QleadsD_AphaseToDaxis  idVec2=[-200, 0, 200] A  iqVec2=[-200, 0, 200] A  magVec2=[0, 100, 200] A  betaVec2=[-180, -90, 0, 90, 180] deg  xVec2=[0, 5, 10, 15, 20, 25, 30] deg  fluxD_dq0=zeros(3, 3, 7) Wb  fluxQ_dq0=zeros(3, 3, 7) Wb  fluxA_dq0=zeros(3, 3, 7) Wb  Torque_dq0=ones(3, 3, 7) N*m  fluxD_IBX=zeros(3, 5, 7) Wb  fluxQ_IBX=zeros(3, 5, 7) Wb  fluxA_IBX=zeros(3, 5, 7) Wb  Torque_IBX=zeros(3, 5, 7) N*m  rotorLossCoeff_k_h_DQ=zeros(3, 3) W/Hz  rotorLossCoeff_k_J_DQ=zeros(3, 3) W/Hz^2  rotorLossCoeff_k_ex_DQ=zeros(3, 3) W/Hz^(3/2)  rotorLossCoeff_k_h_IB=zeros(3, 5) W/Hz  rotorLossCoeff_k_J_IB=zeros(3, 5) W/Hz^2  rotorLossCoeff_k_ex_IB=zeros(3, 5) W/Hz^(3/2)  statorLossCoeff_k_h_DQ=zeros(3, 3) W/Hz  statorLossCoeff_k_J_DQ=zeros(3, 3) W/Hz^2  statorLossCoeff_k_ex_DQ=zeros(3, 3) W/Hz^(3/2)  statorLossCoeff_k_h_IB=zeros(3, 5) W/Hz  statorLossCoeff_k_J_IB=zeros(3, 5) W/Hz^2  statorLossCoeff_k_ex_IB=zeros(3, 5) W/Hz^(3/2)  wVec=[1000, 2000] rpm  rotorLossTable_DQ=zeros(3, 3, 2) W  statorLossTable_DQ=zeros(3, 3, 2) W  rotorLossTable_IB=zeros(3, 5, 2) W  statorLossTable_IB=zeros(3, 5, 2) W  electrical_torque_before_iron_losses_specify=off  electrical_torque_before_iron_losses_priority=None  electrical_torque_before_iron_losses=0 N*m  electrical_torque_before_iron_losses_nominal_specify=off  electrical_torque_before_iron_losses_nominal_value=1  electrical_torque_before_iron_losses_nominal_unit=N*m  Qrotor_specify=off  Qrotor_priority=None  Qrotor=0 J/s  Qrotor_nominal_specify=off  Qrotor_nominal_value=1  Qrotor_nominal_unit=J/s  Qstator_specify=off  Qstator_priority=None  Qstator=0 J/s  Qstator_nominal_specify=off  Qstator_nominal_value=1  Qstator_nominal_unit=J/s
      settings: InternalSimscapePortConfiguration="{\"Bottom\":[],\"Left\":[{\"id\":\"a\",\"label\":\"a\",\"type\":\"foundation.electrical.electrical\"},{\"id\":\"b\",\"label\":\"b\",\"type\":\"foundation.electrical.electrical\"},{\"id\":\"c\",\"label\":\"c\",\"type\":\"foundation.electrical.electrical\"},{\"id\":\"n\",\"label\":\"n\",\"type\":\"foundation.electrical.electrical\"}],\"Right\":[{\"id\":\"R\",\"label\":\"R\",\"type\":\"foundation.mechanical.rotational.rotational\"},{\"id\":\"C\",\"label\":\"C\",\"type\":\"foundation.mechanical.rotational.rotational\"}],\"Top\":[]}"
  Phase Splitter : ee_lib/Connectors & References/Phase Splitter
  ~ : PMIOPort  Side=Left
  neutral : PMIOPort  Port=2  Side=Left
  R : PMIOPort  Port=3  Side=Right
  C : PMIOPort  Port=4  Side=Right
  connections:
  ~/RConn1 -- Phase Splitter/LConn1
  FEM-Parameterized PMSM/LConn1 -- Phase Splitter/RConn1
  FEM-Parameterized PMSM/LConn3 -- Phase Splitter/RConn3
  FEM-Parameterized PMSM/LConn2 -- Phase Splitter/RConn2
  R/RConn1 -- FEM-Parameterized PMSM/RConn1
  C/RConn1 -- FEM-Parameterized PMSM/RConn2
  neutral/RConn1 -- FEM-Parameterized PMSM/LConn4

== system e11_pmsm_nonlin_fwc/Inverter and Motor/Motor Model/Non-linear PMSM with 2D LUTs ==
  PMSM : ee_lib/Electromechanical/Permanent Magnet/PMSM  port_option=ee.enum.threePhasePort.composite  winding_type=ee.enum.statorconnection.wye  machine_param=ee.enum.pmsm.parameterization.tabulated  nPolePairs=pmsm.p  pmflux_param=ee.enum.pmflux.fluxlinkage  pm_flux_linkage=0.03 Wb  torque_constant=0.18 N*m/A  back_emf_constant=0.18 V*s/rad  stator_param=ee.enum.statorparam.LdLqL0  Ld=0.00019 H  Lq=0.00025 H  idVec=PMSMLUT.idVec A  iqVec=PMSMLUT.iqVec A  LdMatrix=PMSMLUT.LdTable H  LqMatrix=PMSMLUT.LqTable H  PmMatrix=PMSMLUT.FluxPMTable Wb  ktMatrix=0.18 * ones(3, 3) N*m/A  keMatrix=0.18 * ones(3, 3) V*s/rad  L0=0.00016 H  Ls=0.0002 H  Lm=-0.00002 H  Ms=0.00002 H  Rs=pmsm.Rs Ohm  zero_sequence=ee.enum.park.zerosequence.include  axes_param=ee.enum.rotorangle.daxis  loss_param=ee.enum.ironloss.none  losses_oc=[0, 0, 0] W  losses_sc=[0, 0, 0] W  f_losses=60 Hz  Isc_losses=95 A  J=pmsm.J kg*m^2  lam=pmsm.B N*m*s/rad  i_d_specify=off  i_d_priority=None  i_d=0 A  i_d_nominal_specify=off  i_d_nominal_value=1  i_d_nominal_unit=A  i_q_specify=off  i_q_priority=None  i_q=0 A  i_q_nominal_specify=off  i_q_nominal_value=1  i_q_nominal_unit=A  torque_specify=off  torque_priority=None  torque=0 N*m  torque_nominal_specify=off  torque_nominal_value=1  torque_nominal_unit=N*m  angular_velocity_specify=on  angular_velocity_priority=None  angular_velocity=0 rpm  angular_velocity_nominal_specify=off  angular_velocity_nominal_value=1  angular_velocity_nominal_unit=rpm  angular_position_specify=on  angular_position_priority=None  angular_position=0 deg  angular_position_nominal_specify=off  angular_position_nominal_value=1  angular_position_nominal_unit=deg  alpha=3.93e-3 1/K  alpha_flux=-0.001 1/K  Tmeas=298.15 K  stator_thermal_mass=100 J/K  rotor_thermal_mass=200 J/K  Rm_percent_rotor=90  Rd_percent_rotor=30  temperatureA_specify=off  temperatureA_priority=High  temperatureA=25 degC  temperatureA_nominal_specify=off  temperatureA_nominal_value=1  temperatureA_nominal_unit=degC  temperatureB_specify=off  temperatureB_priority=High  temperatureB=25 degC  temperatureB_nominal_specify=off  temperatureB_nominal_value=1  temperatureB_nominal_unit=degC  temperatureC_specify=off  temperatureC_priority=High  temperatureC=25 degC  temperatureC_nominal_specify=off  temperatureC_nominal_value=1  temperatureC_nominal_unit=degC  temperatureR_specify=off  temperatureR_priority=High  temperatureR=25 degC  temperatureR_nominal_specify=off  temperatureR_nominal_value=1  temperatureR_nominal_unit=degC
      settings: InternalSimscapePortConfiguration="{\"Bottom\":[],\"Left\":[{\"id\":\"N\",\"label\":\"~\",\"type\":\"foundation.electrical.three_phase\"},{\"id\":\"n\",\"label\":\"n\",\"type\":\"foundation.electrical.electrical\"}],\"Right\":[{\"id\":\"R\",\"label\":\"R\",\"type\":\"foundation.mechanical.rotational.rotational\"},{\"id\":\"C\",\"label\":\"C\",\"type\":\"foundation.mechanical.rotational.rotational\"}],\"Top\":[]}"
  ~ : PMIOPort  Side=Left
  neutral : PMIOPort  Port=2  Side=Left
  R : PMIOPort  Port=3  Side=Right
  C : PMIOPort  Port=4  Side=Right
  connections:
  PMSM/LConn1 -- ~/RConn1
  PMSM/LConn2 -- neutral/RConn1
  PMSM/RConn1 -- R/RConn1
  PMSM/RConn2 -- C/RConn1

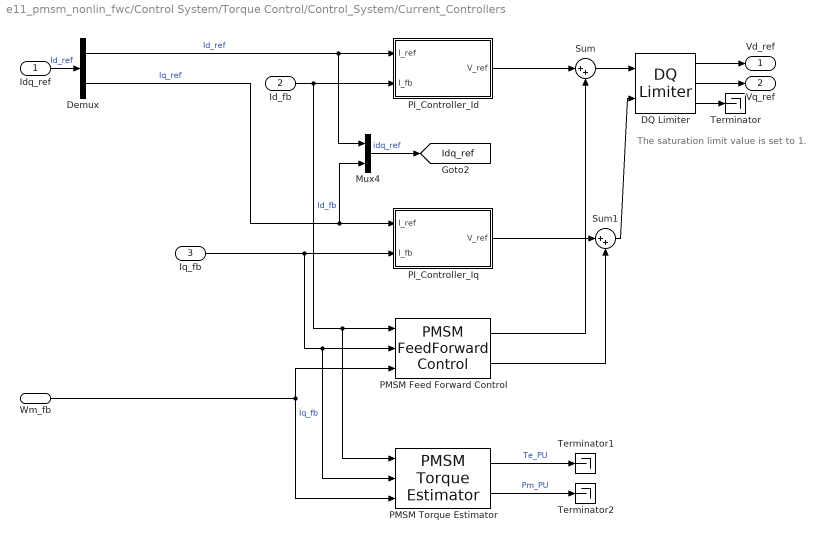
== system e11_pmsm_nonlin_fwc/Control System/Torque Control/Control_System/Current_Controllers ==
  note: The saturation limit value is set to 1.
  Idq_ref : Inport
  Id_fb : Inport  Port=2
  Iq_fb : Inport  Port=3
  Wm_fb : Inport  Port=4
  DQ Limiter : mcbcontrolslib/DQ Limiter  satMethodInputType=Specify via dialog  satMethodSelected=D-Q equivalence  satLimitInputType=Specify via dialog  Vmax=1
  Demux : Demux  Outputs=2
  Mux4 : Mux  Inputs=2
  PI_Controller_Id : Subsystem
  PI_Controller_Iq : Subsystem
  PMSM Feed Forward Control : mcbpmsmnonlinearlib/PMSM FeedForward Control  polePairs=pmsm.p  nonLinearityChoice=Non-linear model with Ld, Lq, and FluxPM LUTs  Ld=pmsm.Ld  Lq=pmsm.Lq  FluxPM=pmsm.FluxPM  idVec=PMSMLUT.idVec  iqVec=PMSMLUT.iqVec  LdTable=PMSMLUT.LdTable  LqTable=PMSMLUT.LqTable  FluxPMTable=PMSMLUT.FluxPMTable  FluxDTable=[-1.6,-1.6,-1.6,-1.6,-1.6;2.4,2.4,2.4,2.4,2.4;6.4,6.4,6.4,6.4,6.4;10.4,10.4,10.4,10.4,10.4]*1e-3  FluxQTable=[-8,-4,0,4,8;-8,-4,0,4,8;-8,-4,0,4,8;-8,-4,0,4,8]*1e-3  Vsat_input_select=Specify via dialog  v_sat=0.05*PU_System.V_base  Units=Per-Unit (PU)  V_base=PU_System.V_base  I_base=PU_System.I_base  N_base=PU_System.N_base  scaledTables=on
  PMSM Torque Estimator : mcbpmsmnonlinearlib/PMSM Torque Estimator  polePairs=pmsm.p  nonLinearityChoice=Non-linear model with Ld, Lq, and FluxPM LUTs  Ld=pmsm.Ld  Lq=pmsm.Lq  FluxPM=pmsm.FluxPM  idVec=PMSMLUT.idVec  iqVec=PMSMLUT.iqVec  LdTable=PMSMLUT.LdTable  LqTable=PMSMLUT.LqTable  FluxPMTable=PMSMLUT.FluxPMTable  FluxDTable=[-1.6,-1.6,-1.6,-1.6,-1.6;2.4,2.4,2.4,2.4,2.4;6.4,6.4,6.4,6.4,6.4;10.4,10.4,10.4,10.4,10.4]*1e-3  FluxQTable=[-8,-4,0,4,8;-8,-4,0,4,8;-8,-4,0,4,8;-8,-4,0,4,8]*1e-3  Units=Per-Unit (PU)  V_base=PU_System.V_base  I_base=PU_System.I_base  N_base=PU_System.N_base  T_base=5.46  P_base=3464.1016  scaledTables=on
  Sum : Sum  Inputs=|++
  Sum1 : Sum  Inputs=|++
  Terminator : Terminator
  Terminator1 : Terminator
  Terminator2 : Terminator
  Vd_ref : Outport  VectorParamsAs1DForOutWhenUnconnected=off
  Vq_ref : Outport  Port=2  VectorParamsAs1DForOutWhenUnconnected=off
  tag scope: Idq_ref=global
  wires:
  Id_fb/1 -> PMSM Torque Estimator/1, PMSM Feed Forward Control/1, PI_Controller_Id/2(I_fb)  "Id_fb"
  DQ Limiter/1 -> Vd_ref/1
  DQ Limiter/2 -> Vq_ref/1
  PI_Controller_Id/1(V_ref) -> Sum/1
  PMSM Torque Estimator/1 -> Terminator1/1  "Te_PU"
  Iq_fb/1 -> PMSM Torque Estimator/2, PMSM Feed Forward Control/2, PI_Controller_Iq/2(I_fb)  "Iq_fb"
  PI_Controller_Iq/1(V_ref) -> Sum1/1
  Sum1/1 -> DQ Limiter/2
  Sum/1 -> DQ Limiter/1
  DQ Limiter/3 -> Terminator/1
  PMSM Feed Forward Control/1 -> Sum/2
  PMSM Feed Forward Control/2 -> Sum1/2
  Idq_ref/1 -> Demux/1  "Id_ref"
  PMSM Torque Estimator/2 -> Terminator2/1  "Pm_PU"
  Wm_fb/1 -> PMSM Torque Estimator/3, PMSM Feed Forward Control/3
  Demux/1 -> Mux4/1, PI_Controller_Id/1(I_ref)  "Id_ref"
  Demux/2 -> Mux4/2, PI_Controller_Iq/1(I_ref)  "Iq_ref"
  Mux4/1 -> [Idq_ref]  "idq_ref"

== system e11_pmsm_nonlin_fwc/Control System/Torque Control/Subsystem/Get_PU  ==
  rad : Inport
  Constant2 : Constant  Value=2*pi  OutDataTypeStr=single  SampleTime=-1
  Get_PU : Gain  Gain=1/(2*pi)  RndMeth=Simplest  OutDataTypeStr=Inherit: Same as input
  Mod : Math  Operator=mod
  PU : Outport  VectorParamsAs1DForOutWhenUnconnected=off
  wires:
  rad/1 -> Mod/1
  Constant2/1 -> Mod/2
  Mod/1 -> Get_PU/1
  Get_PU/1 -> PU/1
